simulink model "sslab"  (R2026b)
settings: Solver=ode45  EnableMultiTasking=on
values from neighbouring files (symbols this model uses):
  Ao = [ 1.38   -0.2077  6.715 -5.676 ... (first row only)    [sslabsc.m]
  Bo = [0 0; 5.679 0; 1.136 -3.146; 1.136 0]    [sslabsc.m]
  Co = [1 0 0 0; 0 1 0 0; 0 0 1 -1]    [sslabsc.m]
  Do = zeros(3,2)    [sslabsc.m]
  K = Kaug(:,1:n)    [acs317.m]
  ki = -Kaug(:,n+1:n+q)    [acs317.m]
  kr = ku + K*kx    [acs317.m]
  x0 = [0.2; 0.1; -0.11; -0.19]    [sslabsc.m]
settings Model: ExtModeTrigMode=oneshot  Creator=bjones  LastModifiedBy=vishy
settings DataIOCC: ReturnWorkspaceOutputs=off  SaveFormat=Array  SignalLoggingSaveFormat=ModelDataLogs
settings OptimizationCC: BlockReduction=off  BooleanDataType=off  LifeSpan=inf  MemsetInitFltsAndDblsToZero=off
settings DebuggingCC: ArithmeticOperatorsInVariantConditions=warning  FcnCallInpInsideContextMsg=warning  MergeDetectMultiDrivingBlocksExec=none  MultiTaskCondExecSysMsg=none  MultiTaskDSMMsg=warning  SFExecutionAtInitializationDiag=none  SFNoUnconditionalDefaultTransitionDiag=warning  SFUnexpectedBacktrackingDiag=warning  SaveWithParameterizedLinksMsg=none  SignalResolutionControl=TryResolveAllWithWarning  StateNameClashWarn=warning  UnderspecifiedInitializationDetection=Classic
settings HardwareCC: ProdEndianess=Unspecified  ProdHWDeviceType=32-bit Generic  ProdIntDivRoundTo=Undefined  ProdLargestAtomicFloat=None  TargetUnknown=on
settings ModelReferenceCC: PropagateSignalLabelsOutOfModel=off
settings SFSimCC: CustomCodeUndefinedFunction=UseInterfaceOnly  SimUseLocalCustomCode=off
settings RTWCC: DLArmComputeVersion=19.05  RTWUseLocalCustomCode=off
settings CodeAppCC: StateflowObjectComments=on
settings GRTTargetCC: CombineOutputUpdateFcns=off  CompOptLevelCompliant=off  GRTInterface=on  MatFileLogging=off  ModelReferenceCompliant=off  ParMdlRefBuildCompliant=off  TargetFcnLib=ansi_tfl_tmw.mat  TargetLangStandard=C89/C90 (ANSI)
settings ConfigComp: CovExternalEMLEnable=off  CovSaveCumulativeToWorkspaceVar=on  CovSaveSingleToWorkspaceVar=on

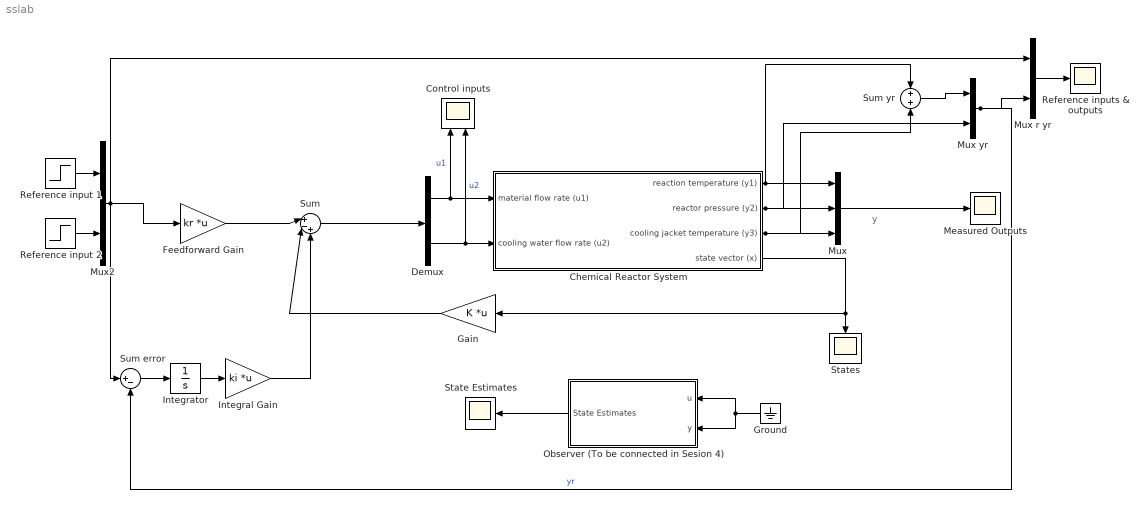
== system sslab ==
  note: y
  Chemical Reactor System : Subsystem  mask(System Block){}
      mask help: Chemical reactor system used for the ACS6004 laboratory. Please ask a demonstrator or press help if you are interested in the underlying workings of the system.
      mask Help:
      | This is the chemical reactor system block for use in the ACS6004 laboratory. This block implements a continuous time state space model of the system, using a set of pre-defined system matrices found in the sslabsc.m file.
      | 
      | This block should not be edited, and for further information about the block please ask a demonstrator.
  Control inputs : Scope  NumInputPorts=2
      settings: ActiveDisplayYMinimum=-5  ActiveDisplayYMaximum=5
  Demux : Demux  Outputs=2
  Feedforward Gain : Gain  Gain=kr  Multiplication=Matrix(K*u)
  Gain : Gain  Gain=K  Multiplication=Matrix(K*u)
  Ground : Ground
  Integral Gain : Gain  Gain=ki  Multiplication=Matrix(K*u)
  Integrator : Integrator
  Measured Outputs : Scope
      settings: ActiveDisplayYMinimum=-3.2585684143948816E+7  ActiveDisplayYMaximum=1.5433148424444228E+8
  Mux : Mux  Inputs=3
  Mux r yr : Mux  Inputs=2
  Mux yr : Mux  Inputs=2
  Mux2 : Mux  Inputs=2
  "Observer (To be connected in Sesion 4) " : Subsystem
  Reference input 1 : Step  SampleTime=0
  Reference input 2 : Step  Time=2  FinalValue=1.5  SampleTime=0
  Reference inputs & outputs : Scope
  State Estimates : Scope
  States : Scope
  Sum : Sum  Inputs=|+-+  RndMeth=Round
  Sum error : Sum  Inputs=|+-
  Sum yr : Sum
  wires:
  Reference input 1/1 -> Mux2/1
  Reference input 2/1 -> Mux2/2
  Chemical Reactor System/4(state vector (x)) -> States/1, Gain/1
  Chemical Reactor System/1(reaction temperature (y1)) -> Mux/1, Sum yr/1
  Chemical Reactor System/2(reactor pressure (y2)) -> Mux/2, Mux yr/2
  Chemical Reactor System/3(cooling jacket temperature (y3)) -> Mux/3, Sum yr/2
  Mux/1 -> Measured Outputs/1
  Demux/1 -> Chemical Reactor System/1(material flow rate (u1)), Control inputs/1  "u1"
  Demux/2 -> Chemical Reactor System/2(cooling water flow rate (u2)), Control inputs/2  "u2"
  "Observer (To be connected in Sesion 4) "/1(State Estimates) -> State Estimates/1
  Ground/1 -> "Observer (To be connected in Sesion 4) "/1(u), "Observer (To be connected in Sesion 4) "/2(y)
  Sum/1 -> Demux/1
  Gain/1 -> Sum/2
  Mux2/1 -> Feedforward Gain/1, Mux r yr/1, Sum error/1
  Feedforward Gain/1 -> Sum/1
  Sum yr/1 -> Mux yr/1
  Mux yr/1 -> Mux r yr/2, Sum error/2  "yr"
  Mux r yr/1 -> Reference inputs & outputs/1
  Sum error/1 -> Integrator/1
  Integrator/1 -> Integral Gain/1
  Integral Gain/1 -> Sum/3

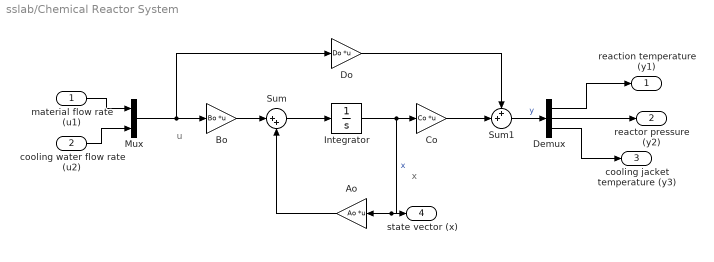
== system sslab/Chemical Reactor System ==
  note: u
  note: x
  material flow rate (u1) : Inport
  cooling water flow rate (u2) : Inport  Port=2
  Ao : Gain  Gain=Ao  Multiplication=Matrix(K*u)  SaturateOnIntegerOverflow=on  OutDataTypeStr=Inherit: Same as input  ParamDataTypeStr=Inherit: Same as input
  Bo : Gain  Gain=Bo  Multiplication=Matrix(K*u)  SaturateOnIntegerOverflow=on  OutDataTypeStr=Inherit: Same as input  ParamDataTypeStr=Inherit: Same as input
  Co : Gain  Gain=Co  Multiplication=Matrix(K*u)  SaturateOnIntegerOverflow=on  OutDataTypeStr=Inherit: Same as input  ParamDataTypeStr=Inherit: Same as input
  Demux : Demux  Outputs=3
  Do : Gain  Gain=Do  Multiplication=Matrix(K*u)  SaturateOnIntegerOverflow=on  OutDataTypeStr=Inherit: Same as input  ParamDataTypeStr=Inherit: Same as input
  Integrator : Integrator  InitialCondition=x0
  Mux : Mux  Inputs=2
  Sum : Sum  Inputs=|++  InputSameDT=on  SaturateOnIntegerOverflow=on  OutDataTypeStr=Inherit: Same as first input
  Sum1 : Sum  Inputs=++|  InputSameDT=on  SaturateOnIntegerOverflow=on  OutDataTypeStr=Inherit: Same as first input
  reaction temperature (y1) : Outport  VectorParamsAs1DForOutWhenUnconnected=off
  reactor pressure (y2) : Outport  Port=2  VectorParamsAs1DForOutWhenUnconnected=off
  cooling jacket temperature (y3) : Outport  Port=3  VectorParamsAs1DForOutWhenUnconnected=off
  state vector (x) : Outport  Port=4  VectorParamsAs1DForOutWhenUnconnected=off
  wires:
  Integrator/1 -> Co/1, Ao/1, state vector (x)/1  "x"
  Sum/1 -> Integrator/1
  Bo/1 -> Sum/1
  Ao/1 -> Sum/2
  Do/1 -> Sum1/1
  Co/1 -> Sum1/2
  Mux/1 -> Bo/1, Do/1
  material flow rate (u1)/1 -> Mux/1
  cooling water flow rate (u2)/1 -> Mux/2
  Sum1/1 -> Demux/1  "y"
  Demux/1 -> reaction temperature (y1)/1
  Demux/2 -> reactor pressure (y2)/1
  Demux/3 -> cooling jacket temperature (y3)/1

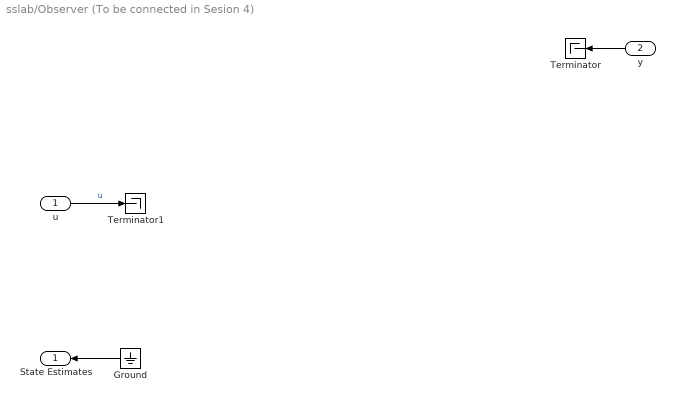
== system sslab/Observer (To be connected in Sesion 4)  ==
  u : Inport
  y : Inport  Port=2
  Ground : Ground
  Terminator : Terminator
  Terminator1 : Terminator
  State Estimates : Outport  VectorParamsAs1DForOutWhenUnconnected=off
  wires:
  y/1 -> Terminator/1
  u/1 -> Terminator1/1  "u"
  Ground/1 -> State Estimates/1
